simulink model "SNS_Li_CPG"  (R2025a)
settings: Solver=ode45  StartTime=0.0  StopTime=30  MaxStep=1e-3  RelTol=1e-3
libraries: SNS_Library x134
settings Model: Creator=Ben Bolen  LastModifiedBy=Ben Bolen

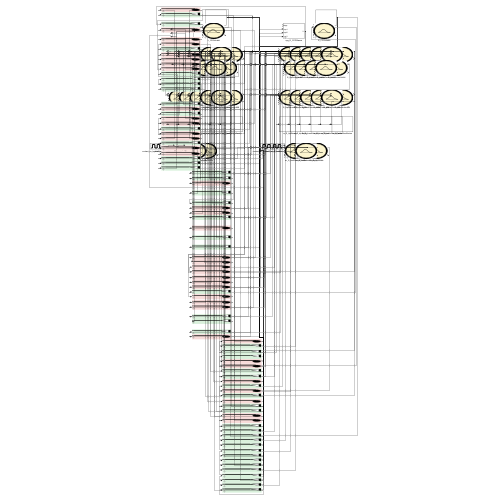
[thumbnail: Simulink's stored preview of the top-level diagram]
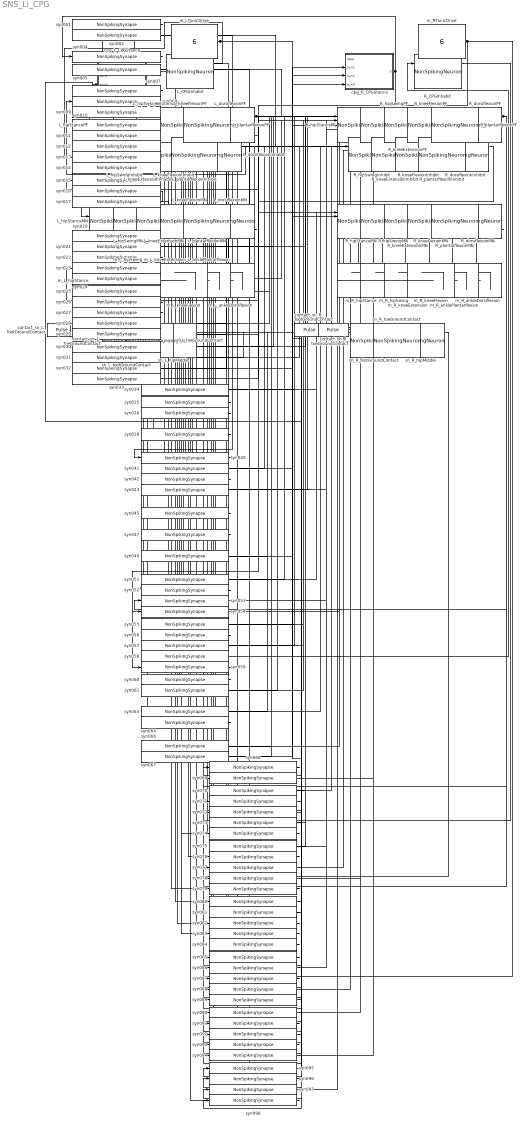
== system SNS_Li_CPG ==
  L_CPGInhabit : SNS_Library/NonSpikingNeuron  Vrest=-52  Gm=0.12  Cm=5  Thr=-50  Slope=1
  L_dorsiflexionInhabit : SNS_Library/NonSpikingNeuron  Vrest=-52  Gm=0.12  Cm=5  Thr=-50  Slope=1
  L_dorsiflexionMN : SNS_Library/NonSpikingNeuron  Vrest=-52  Gm=0.5  Cm=5  Thr=-45  Slope=1
  L_dorsiflexionPF : SNS_Library/NonSpikingNeuron  Vrest=-52  Gm=0.12  Cm=5  Thr=-50  Slope=1
  L_hipStanceMN : SNS_Library/NonSpikingNeuron  Vrest=-52  Gm=0.5  Cm=5  Thr=-45  Slope=1
  L_hipStancePF : SNS_Library/NonSpikingNeuron  Vrest=-52  Gm=0.12  Cm=5  Thr=-50  Slope=1
  L_hipSwingInhibit : SNS_Library/NonSpikingNeuron  Vrest=-52  Gm=0.12  Cm=5  Thr=-50  Slope=1
  L_hipSwingMN : SNS_Library/NonSpikingNeuron  Vrest=-52  Gm=0.5  Cm=5  Thr=-45  Slope=1
  L_hipSwingPF : SNS_Library/NonSpikingNeuron  Vrest=-52  Gm=0.12  Cm=5  Thr=-50  Slope=1
  L_kneeExtensionInhabit : SNS_Library/NonSpikingNeuron  Vrest=-52  Gm=0.12  Cm=5  Thr=-50  Slope=1
  L_kneeExtensionMN : SNS_Library/NonSpikingNeuron  Vrest=-52  Gm=0.5  Cm=5  Thr=-45  Slope=1
  L_kneeExtensionPF : SNS_Library/NonSpikingNeuron  Vrest=-52  Gm=0.12  Cm=5  Thr=-50  Slope=1
  L_kneeFlexionInhibit : SNS_Library/NonSpikingNeuron  Vrest=-52  Gm=0.12  Cm=5  Thr=-50  Slope=1
  L_kneeFlexionMN : SNS_Library/NonSpikingNeuron  Vrest=-52  Gm=0.5  Cm=5  Thr=-45  Slope=1
  L_kneeFlexionPF : SNS_Library/NonSpikingNeuron  Vrest=-52  Gm=0.12  Cm=5  Thr=-50  Slope=1
  L_plantarflexionInhibit : SNS_Library/NonSpikingNeuron  Vrest=-52  Gm=0.12  Cm=5  Thr=-50  Slope=1
  L_plantarflexionMN : SNS_Library/NonSpikingNeuron  Vrest=-52  Gm=0.5  Cm=5  Thr=-45  Slope=1
  L_plantarflexionPF : SNS_Library/NonSpikingNeuron  Vrest=-52  Gm=0.12  Cm=5  Thr=-50  Slope=1
  R_CPGInhabit : SNS_Library/NonSpikingNeuron  Vrest=-52  Gm=0.12  Cm=5  Thr=-50  Slope=1
  R_dorsiflexionInhibit : SNS_Library/NonSpikingNeuron  Vrest=-52  Gm=0.12  Cm=5  Thr=-50  Slope=1
  R_dorsiflexionMN : SNS_Library/NonSpikingNeuron  Vrest=-52  Gm=0.5  Cm=5  Thr=-45  Slope=1
  R_dorsiflexionPF : SNS_Library/NonSpikingNeuron  Vrest=-52  Gm=0.12  Cm=5  Thr=-50  Slope=1
  R_hipStanceMN : SNS_Library/NonSpikingNeuron  Vrest=-52  Gm=0.5  Cm=5  Thr=-45  Slope=1
  R_hipStancePF : SNS_Library/NonSpikingNeuron  Vrest=-52  Gm=0.12  Cm=5  Thr=-50  Slope=1
  R_hipSwingInhibit : SNS_Library/NonSpikingNeuron  Vrest=-52  Gm=0.12  Cm=5  Thr=-50  Slope=1
  R_hipSwingMN : SNS_Library/NonSpikingNeuron  Vrest=-52  Gm=0.5  Cm=5  Thr=-45  Slope=1
  R_hipSwingPF : SNS_Library/NonSpikingNeuron  Vrest=-52  Gm=0.12  Cm=5  Thr=-50  Slope=1
  R_kneeExtensionInhibit : SNS_Library/NonSpikingNeuron  Vrest=-52  Gm=0.12  Cm=5  Thr=-50  Slope=1
  R_kneeExtensionMN : SNS_Library/NonSpikingNeuron  Vrest=-52  Gm=0.5  Cm=5  Thr=-45  Slope=1
  R_kneeExtensionPF : SNS_Library/NonSpikingNeuron  Vrest=-52  Gm=0.12  Cm=5  Thr=-50  Slope=1
  R_kneeFlexionInhibit : SNS_Library/NonSpikingNeuron  Vrest=-52  Gm=0.12  Cm=5  Thr=-50  Slope=1
  R_kneeFlexionMN : SNS_Library/NonSpikingNeuron  Vrest=-52  Gm=0.5  Cm=5  Thr=-45  Slope=1
  R_kneeFlexionPF : SNS_Library/NonSpikingNeuron  Vrest=-52  Gm=0.12  Cm=5  Thr=-50  Slope=1
  R_plantarflexionInhibit : SNS_Library/NonSpikingNeuron  Vrest=-52  Gm=0.12  Cm=5  Thr=-50  Slope=1
  R_plantarflexionMN : SNS_Library/NonSpikingNeuron  Vrest=-52  Gm=0.5  Cm=5  Thr=-45  Slope=1
  R_plantarflexionPF : SNS_Library/NonSpikingNeuron  Vrest=-52  Gm=0.12  Cm=5  Thr=-50  Slope=1
  contact_sn_L_footGroundContact : DiscretePulseGenerator  PulseType=Time based  Amplitude=10  PulseWidth=35
  contact_sn_L_toeGroundContact : DiscretePulseGenerator  PulseType=Time based  Amplitude=10  PulseWidth=35
  contact_sn_R_footGroundContact : DiscretePulseGenerator  PulseType=Time based  Amplitude=10  PulseWidth=35  PhaseDelay=1
  contact_sn_R_toeGroundContact : DiscretePulseGenerator  PulseType=Time based  Amplitude=10  PulseWidth=35  PhaseDelay=1
  cpg_L_CPGStance : Subsystem
      mask help: Li stance CPG v1 (ADAPTATION): graded cell + slow Adp burst termination, tau = documented tau_Ca 7.5 s. Ports: 1 Iapp (nA currents), 2-4 synaptic inputs, out = cell V (mV).
  cpg_R_CPGStance : Subsystem
      mask help: Li stance CPG v1 (ADAPTATION): graded cell + slow Adp burst termination, tau = documented tau_Ca 7.5 s. Ports: 1 Iapp (nA currents), 2-4 synaptic inputs, out = cell V (mV).
  in_LTonicDrive : Constant  Value=6
  in_RTonicDrive : Constant  Value=6
  m_L_ankleDorsiflexion : Terminator
  m_L_anklePlantarflexion : Terminator
  m_L_hipStance : Terminator
  m_L_hipSwing : Terminator
  m_L_kneeExtension : Terminator
  m_L_kneeFlexion : Terminator
  m_R_ankleDorsiflexion : Terminator
  m_R_anklePlantarflexion : Terminator
  m_R_hipStance : Terminator
  m_R_hipSwing : Terminator
  m_R_kneeExtension : Terminator
  m_R_kneeFlexion : Terminator
  sn_L_footGroundContact : SNS_Library/NonSpikingNeuron  Vrest=-52  Gm=0.12  Cm=2  Thr=-55  Slope=1
  sn_L_hipMiddle : SNS_Library/NonSpikingNeuron  Vrest=-52  Gm=0.12  Cm=5  Thr=-50  Slope=1
  sn_L_toeGroundContact : SNS_Library/NonSpikingNeuron  Vrest=-52  Gm=0.12  Cm=2  Thr=-55  Slope=1
  sn_R_footGroundContact : SNS_Library/NonSpikingNeuron  Vrest=-52  Gm=0.12  Cm=2  Thr=-55  Slope=1
  sn_R_hipMiddle : SNS_Library/NonSpikingNeuron  Vrest=-52  Gm=0.12  Cm=5  Thr=-50  Slope=1
  sn_R_toeGroundContact : SNS_Library/NonSpikingNeuron  Vrest=-52  Gm=0.12  Cm=2  Thr=-55  Slope=1
  syn001 : SNS_Library/NonSpikingSynapse  gmax=1  Esyn=-72  ThrPre=-50  SlopePre=1
  syn002 : SNS_Library/NonSpikingSynapse  gmax=8  Esyn=0  ThrPre=-50  SlopePre=1
  syn004 : SNS_Library/NonSpikingSynapse  gmax=1  Esyn=0  ThrPre=-50  SlopePre=1
  syn005 : SNS_Library/NonSpikingSynapse  gmax=1  Esyn=-72  ThrPre=-50  SlopePre=1
  syn007 : SNS_Library/NonSpikingSynapse  gmax=1  Esyn=-72  ThrPre=-50  SlopePre=1
  syn008 : SNS_Library/NonSpikingSynapse  gmax=1  Esyn=-72  ThrPre=-50  SlopePre=1
  syn009 : SNS_Library/NonSpikingSynapse  gmax=1  Esyn=0  ThrPre=-50  SlopePre=1
  syn010 : SNS_Library/NonSpikingSynapse  gmax=1  Esyn=-72  ThrPre=-50  SlopePre=1
  syn011 : SNS_Library/NonSpikingSynapse  gmax=1  Esyn=-72  ThrPre=-50  SlopePre=1
  syn012 : SNS_Library/NonSpikingSynapse  gmax=1  Esyn=-72  ThrPre=-50  SlopePre=1
  syn013 : SNS_Library/NonSpikingSynapse  gmax=1  Esyn=-72  ThrPre=-50  SlopePre=1
  syn014 : SNS_Library/NonSpikingSynapse  gmax=8  Esyn=0  ThrPre=-50  SlopePre=1
  syn015 : SNS_Library/NonSpikingSynapse  gmax=1  Esyn=0  ThrPre=-50  SlopePre=1
  syn016 : SNS_Library/NonSpikingSynapse  gmax=1  Esyn=0  ThrPre=-50  SlopePre=1
  syn017 : SNS_Library/NonSpikingSynapse  gmax=1  Esyn=0  ThrPre=-50  SlopePre=1
  syn020 : SNS_Library/NonSpikingSynapse  gmax=1  Esyn=0  ThrPre=-50  SlopePre=1
  syn021 : SNS_Library/NonSpikingSynapse  gmax=1  Esyn=-72  ThrPre=-50  SlopePre=1
  syn022 : SNS_Library/NonSpikingSynapse  gmax=1  Esyn=0  ThrPre=-50  SlopePre=1
  syn023 : SNS_Library/NonSpikingSynapse  gmax=1  Esyn=-72  ThrPre=-50  SlopePre=1
  syn024 : SNS_Library/NonSpikingSynapse  gmax=1  Esyn=-72  ThrPre=-50  SlopePre=1
  syn025 : SNS_Library/NonSpikingSynapse  gmax=1  Esyn=0  ThrPre=-50  SlopePre=1
  syn026 : SNS_Library/NonSpikingSynapse  gmax=1  Esyn=-72  ThrPre=-50  SlopePre=1
  syn027 : SNS_Library/NonSpikingSynapse  gmax=1  Esyn=-72  ThrPre=-50  SlopePre=1
  syn028 : SNS_Library/NonSpikingSynapse  gmax=2  Esyn=0  ThrPre=-50  SlopePre=1
  syn029 : SNS_Library/NonSpikingSynapse  gmax=1  Esyn=-72  ThrPre=-50  SlopePre=1
  syn030 : SNS_Library/NonSpikingSynapse  gmax=1  Esyn=-72  ThrPre=-50  SlopePre=1
  syn031 : SNS_Library/NonSpikingSynapse  gmax=5  Esyn=0  ThrPre=-50  SlopePre=1
  syn032 : SNS_Library/NonSpikingSynapse  gmax=1  Esyn=0  ThrPre=-50  SlopePre=1
  syn033 : SNS_Library/NonSpikingSynapse  gmax=1  Esyn=0  ThrPre=-50  SlopePre=1
  syn034 : SNS_Library/NonSpikingSynapse  gmax=1  Esyn=0  ThrPre=-50  SlopePre=1
  syn035 : SNS_Library/NonSpikingSynapse  gmax=1  Esyn=0  ThrPre=-50  SlopePre=1
  syn036 : SNS_Library/NonSpikingSynapse  gmax=1  Esyn=-72  ThrPre=-50  SlopePre=1
  syn038 : SNS_Library/NonSpikingSynapse  gmax=5  Esyn=0  ThrPre=-50  SlopePre=1
  syn040 : SNS_Library/NonSpikingSynapse  gmax=8  Esyn=0  ThrPre=-50  SlopePre=1
  syn041 : SNS_Library/NonSpikingSynapse  gmax=1  Esyn=-72  ThrPre=-50  SlopePre=1
  syn042 : SNS_Library/NonSpikingSynapse  gmax=1  Esyn=-72  ThrPre=-50  SlopePre=1
  syn043 : SNS_Library/NonSpikingSynapse  gmax=1  Esyn=0  ThrPre=-50  SlopePre=1
  syn045 : SNS_Library/NonSpikingSynapse  gmax=1  Esyn=-72  ThrPre=-50  SlopePre=1
  syn047 : SNS_Library/NonSpikingSynapse  gmax=6  Esyn=0  ThrPre=-50  SlopePre=1
  syn049 : SNS_Library/NonSpikingSynapse  gmax=4  Esyn=0  ThrPre=-50  SlopePre=1
  syn051 : SNS_Library/NonSpikingSynapse  gmax=1  Esyn=-72  ThrPre=-50  SlopePre=1
  syn052 : SNS_Library/NonSpikingSynapse  gmax=1  Esyn=-72  ThrPre=-50  SlopePre=1
  syn053 : SNS_Library/NonSpikingSynapse  gmax=1  Esyn=-72  ThrPre=-50  SlopePre=1
  syn054 : SNS_Library/NonSpikingSynapse  gmax=1  Esyn=-72  ThrPre=-50  SlopePre=1
  syn055 : SNS_Library/NonSpikingSynapse  gmax=1  Esyn=-72  ThrPre=-50  SlopePre=1
  syn056 : SNS_Library/NonSpikingSynapse  gmax=1  Esyn=-72  ThrPre=-50  SlopePre=1
  syn057 : SNS_Library/NonSpikingSynapse  gmax=1  Esyn=-72  ThrPre=-50  SlopePre=1
  syn058 : SNS_Library/NonSpikingSynapse  gmax=6  Esyn=0  ThrPre=-50  SlopePre=1
  syn059 : SNS_Library/NonSpikingSynapse  gmax=1  Esyn=-72  ThrPre=-50  SlopePre=1
  syn060 : SNS_Library/NonSpikingSynapse  gmax=1  Esyn=-72  ThrPre=-50  SlopePre=1
  syn061 : SNS_Library/NonSpikingSynapse  gmax=1  Esyn=-72  ThrPre=-50  SlopePre=1
  syn063 : SNS_Library/NonSpikingSynapse  gmax=6  Esyn=0  ThrPre=-50  SlopePre=1
  syn064 : SNS_Library/NonSpikingSynapse  gmax=1  Esyn=0  ThrPre=-50  SlopePre=1
  syn066 : SNS_Library/NonSpikingSynapse  gmax=1  Esyn=0  ThrPre=-50  SlopePre=1
  syn067 : SNS_Library/NonSpikingSynapse  gmax=1  Esyn=-72  ThrPre=-50  SlopePre=1
  syn068 : SNS_Library/NonSpikingSynapse  gmax=1  Esyn=-72  ThrPre=-50  SlopePre=1
  syn069 : SNS_Library/NonSpikingSynapse  gmax=1  Esyn=0  ThrPre=-50  SlopePre=1
  syn070 : SNS_Library/NonSpikingSynapse  gmax=8  Esyn=0  ThrPre=-50  SlopePre=1
  syn071 : SNS_Library/NonSpikingSynapse  gmax=1  Esyn=0  ThrPre=-50  SlopePre=1
  syn072 : SNS_Library/NonSpikingSynapse  gmax=1  Esyn=-72  ThrPre=-50  SlopePre=1
  syn073 : SNS_Library/NonSpikingSynapse  gmax=1  Esyn=-72  ThrPre=-50  SlopePre=1
  syn074 : SNS_Library/NonSpikingSynapse  gmax=8  Esyn=0  ThrPre=-50  SlopePre=1
  syn075 : SNS_Library/NonSpikingSynapse  gmax=1  Esyn=0  ThrPre=-50  SlopePre=1
  syn076 : SNS_Library/NonSpikingSynapse  gmax=1  Esyn=-72  ThrPre=-50  SlopePre=1
  syn077 : SNS_Library/NonSpikingSynapse  gmax=8  Esyn=0  ThrPre=-50  SlopePre=1
  syn078 : SNS_Library/NonSpikingSynapse  gmax=1  Esyn=-72  ThrPre=-50  SlopePre=1
  syn079 : SNS_Library/NonSpikingSynapse  gmax=2  Esyn=0  ThrPre=-50  SlopePre=1
  syn080 : SNS_Library/NonSpikingSynapse  gmax=1  Esyn=-72  ThrPre=-50  SlopePre=1
  syn081 : SNS_Library/NonSpikingSynapse  gmax=6  Esyn=0  ThrPre=-50  SlopePre=1
  syn082 : SNS_Library/NonSpikingSynapse  gmax=4  Esyn=0  ThrPre=-50  SlopePre=1
  syn083 : SNS_Library/NonSpikingSynapse  gmax=1  Esyn=-72  ThrPre=-50  SlopePre=1
  syn084 : SNS_Library/NonSpikingSynapse  gmax=1  Esyn=-72  ThrPre=-50  SlopePre=1
  syn085 : SNS_Library/NonSpikingSynapse  gmax=5  Esyn=0  ThrPre=-50  SlopePre=1
  syn086 : SNS_Library/NonSpikingSynapse  gmax=5  Esyn=0  ThrPre=-50  SlopePre=1
  syn087 : SNS_Library/NonSpikingSynapse  gmax=5  Esyn=0  ThrPre=-50  SlopePre=1
  syn088 : SNS_Library/NonSpikingSynapse  gmax=5  Esyn=0  ThrPre=-50  SlopePre=1
  syn089 : SNS_Library/NonSpikingSynapse  gmax=6  Esyn=0  ThrPre=-50  SlopePre=1
  syn090 : SNS_Library/NonSpikingSynapse  gmax=5  Esyn=0  ThrPre=-50  SlopePre=1
  syn091 : SNS_Library/NonSpikingSynapse  gmax=5  Esyn=0  ThrPre=-50  SlopePre=1
  syn092 : SNS_Library/NonSpikingSynapse  gmax=6  Esyn=0  ThrPre=-50  SlopePre=1
  syn093 : SNS_Library/NonSpikingSynapse  gmax=6  Esyn=0  ThrPre=-50  SlopePre=1
  syn094 : SNS_Library/NonSpikingSynapse  gmax=5  Esyn=0  ThrPre=-50  SlopePre=1
  syn095 : SNS_Library/NonSpikingSynapse  gmax=5  Esyn=0  ThrPre=-50  SlopePre=1
  syn096 : SNS_Library/NonSpikingSynapse  gmax=6  Esyn=0  ThrPre=-50  SlopePre=1
  syn097 : SNS_Library/NonSpikingSynapse  gmax=5  Esyn=0  ThrPre=-50  SlopePre=1
  syn098 : SNS_Library/NonSpikingSynapse  gmax=5  Esyn=0  ThrPre=-50  SlopePre=1
  wires:
  contact_sn_L_footGroundContact/1 -> sn_L_footGroundContact/1
  contact_sn_L_toeGroundContact/1 -> sn_L_toeGroundContact/1
  contact_sn_R_footGroundContact/1 -> sn_R_footGroundContact/1
  contact_sn_R_toeGroundContact/1 -> sn_R_toeGroundContact/1
  L_hipStancePF/1 -> syn001/1, syn016/1, syn027/1, syn079/1
  syn001/1 -> L_hipSwingPF/2
  sn_R_footGroundContact/1 -> syn002/1, syn049/1, syn063/1, syn081/1
  syn002/1 -> R_kneeFlexionInhibit/2
  R_kneeFlexionMN/2 -> m_R_kneeFlexion/1
  cpg_R_CPGStance/1(V) -> syn004/1, syn023/1, syn071/1
  syn004/1 -> L_hipSwingPF/3
  R_kneeExtensionPF/1 -> syn005/1, syn025/1, syn051/1
  syn005/1 -> R_kneeFlexionPF/2
  R_plantarflexionMN/2 -> m_R_anklePlantarflexion/1
  L_kneeExtensionPF/1 -> syn007/1, syn035/1, syn036/1
  syn007/1 -> L_kneeFlexionPF/2
  L_dorsiflexionInhabit/1 -> syn008/1
  syn008/1 -> L_dorsiflexionPF/2
  L_kneeFlexionPF/1 -> syn009/1, syn026/1, syn060/1
  syn009/1 -> L_kneeFlexionMN/2
  L_hipSwingPF/1 -> syn010/1, syn022/1, syn064/1, syn074/1, syn083/1
  syn010/1 -> L_hipStanceMN/2
  R_hipStancePF/1 -> syn011/1, syn028/1, syn029/1, syn032/1
  syn011/1 -> R_hipSwingPF/2
  R_plantarflexionInhibit/1 -> syn012/1
  syn012/1 -> R_plantarflexionPF/2
  L_CPGInhabit/1 -> syn013/1
  syn013/1 -> cpg_L_CPGStance/2(syn1)
  sn_L_footGroundContact/1 -> syn014/1, syn047/1, syn058/1, syn082/1
  syn014/1 -> L_kneeFlexionInhibit/2
  L_dorsiflexionPF/1 -> syn015/1, syn059/1, syn068/1
  syn015/1 -> L_dorsiflexionMN/2
  syn016/1 -> L_hipStanceMN/3
  L_plantarflexionPF/1 -> syn017/1, syn045/1, syn056/1
  syn017/1 -> L_plantarflexionMN/2
  L_hipStanceMN/2 -> m_L_hipStance/1
  L_plantarflexionMN/2 -> m_L_anklePlantarflexion/1
  cpg_L_CPGStance/1(V) -> syn020/1, syn033/1, syn080/1
  syn020/1 -> L_hipStancePF/2
  R_plantarflexionPF/1 -> syn021/1, syn030/1, syn043/1
  syn021/1 -> R_dorsiflexionPF/2
  syn022/1 -> L_hipSwingMN/2
  syn023/1 -> cpg_L_CPGStance/3(syn2)
  R_kneeFlexionInhibit/1 -> syn024/1
  syn024/1 -> R_kneeFlexionPF/3
  syn025/1 -> R_kneeExtensionMN/2
  syn026/1 -> L_kneeExtensionPF/2
  syn027/1 -> L_hipSwingMN/3
  syn028/1 -> R_kneeExtensionPF/2
  syn029/1 -> R_hipSwingMN/2
  syn030/1 -> R_dorsiflexionMN/2
  sn_R_toeGroundContact/1 -> syn031/1
  syn031/1 -> R_dorsiflexionInhibit/2
  syn032/1 -> R_hipStanceMN/2
  syn033/1 -> R_hipSwingPF/3
  R_kneeFlexionPF/1 -> syn034/1, syn055/1, syn057/1
  syn034/1 -> R_kneeFlexionMN/2
  syn035/1 -> L_kneeExtensionMN/2
  syn036/1 -> L_kneeFlexionMN/3
  L_kneeFlexionMN/2 -> m_L_kneeFlexion/1
  sn_L_toeGroundContact/1 -> syn038/1
  syn038/1 -> L_dorsiflexionInhabit/2
  L_dorsiflexionMN/2 -> m_L_ankleDorsiflexion/1
  sn_L_hipMiddle/1 -> syn040/1
  syn040/1 -> L_kneeFlexionInhibit/3
  R_hipSwingInhibit/1 -> syn041/1
  syn041/1 -> R_hipSwingPF/4
  L_kneeFlexionInhibit/1 -> syn042/1
  syn042/1 -> L_kneeFlexionPF/3
  syn043/1 -> R_plantarflexionMN/2
  R_hipStanceMN/2 -> m_R_hipStance/1
  syn045/1 -> L_dorsiflexionPF/3
  L_kneeExtensionMN/2 -> m_L_kneeExtension/1
  syn047/1 -> L_plantarflexionInhibit/2
  R_hipSwingMN/2 -> m_R_hipSwing/1
  syn049/1 -> R_hipSwingInhibit/2
  R_kneeExtensionMN/2 -> m_R_kneeExtension/1
  syn051/1 -> R_kneeFlexionMN/3
  L_hipSwingInhibit/1 -> syn052/1
  syn052/1 -> L_hipSwingPF/4
  R_dorsiflexionPF/1 -> syn053/1, syn069/1, syn078/1
  syn053/1 -> R_plantarflexionPF/3
  R_dorsiflexionInhibit/1 -> syn054/1
  syn054/1 -> R_dorsiflexionPF/3
  syn055/1 -> R_kneeExtensionPF/3
  syn056/1 -> L_dorsiflexionMN/3
  syn057/1 -> R_kneeExtensionMN/3
  syn058/1 -> R_CPGInhabit/2
  syn059/1 -> L_plantarflexionPF/2
  syn060/1 -> L_kneeExtensionMN/3
  R_kneeExtensionInhibit/1 -> syn061/1
  syn061/1 -> R_kneeExtensionPF/4
  L_hipSwingMN/2 -> m_L_hipSwing/1
  syn063/1 -> R_plantarflexionInhibit/2
  syn064/1 -> L_dorsiflexionPF/4
  R_dorsiflexionMN/2 -> m_R_ankleDorsiflexion/1
  R_hipSwingPF/1 -> syn066/1, syn067/1, syn070/1, syn073/1, syn075/1
  syn066/1 -> R_dorsiflexionPF/4
  syn067/1 -> R_hipStancePF/2
  syn068/1 -> L_plantarflexionMN/3
  syn069/1 -> R_dorsiflexionMN/3
  syn070/1 -> R_kneeExtensionInhibit/2
  syn071/1 -> R_hipStancePF/3
  R_CPGInhabit/1 -> syn072/1
  syn072/1 -> cpg_R_CPGStance/2(syn1)
  syn073/1 -> R_hipStanceMN/3
  syn074/1 -> L_kneeExtensionInhabit/2
  syn075/1 -> R_hipSwingMN/3
  L_kneeExtensionInhabit/1 -> syn076/1
  syn076/1 -> L_kneeExtensionPF/3
  sn_R_hipMiddle/1 -> syn077/1
  syn077/1 -> R_kneeFlexionInhibit/3
  syn078/1 -> R_plantarflexionMN/3
  syn079/1 -> L_kneeExtensionPF/4
  syn080/1 -> cpg_R_CPGStance/3(syn2)
  syn081/1 -> L_CPGInhabit/2
  syn082/1 -> L_hipSwingInhibit/2
  syn083/1 -> L_hipStancePF/3
  L_plantarflexionInhibit/1 -> syn084/1
  syn084/1 -> L_plantarflexionPF/3
  in_LTonicDrive/1 -> syn085/1, syn087/1, syn091/1, syn092/1, syn093/1, syn096/1, syn098/1
  syn085/1 -> L_hipSwingPF/5
  in_RTonicDrive/1 -> syn086/1, syn088/1, syn089/1, syn090/1, syn094/1, syn095/1, syn097/1
  syn086/1 -> R_hipSwingPF/5
  syn087/1 -> L_kneeFlexionPF/4
  syn088/1 -> R_kneeFlexionPF/4
  syn089/1 -> cpg_R_CPGStance/4(syn3)
  syn090/1 -> R_plantarflexionPF/4
  syn091/1 -> L_kneeExtensionPF/5
  syn092/1 -> cpg_L_CPGStance/4(syn3)
  syn093/1 -> L_plantarflexionPF/4
  syn094/1 -> R_dorsiflexionPF/5
  syn095/1 -> R_hipStancePF/4
  syn096/1 -> L_dorsiflexionPF/5
  syn097/1 -> R_kneeExtensionPF/5
  syn098/1 -> L_hipStancePF/4

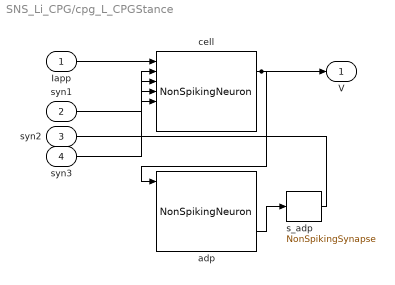
== system SNS_Li_CPG/cpg_L_CPGStance ==
  Iapp : Inport
  syn1 : Inport  Port=2
  syn2 : Inport  Port=3
  syn3 : Inport  Port=4
  adp : SNS_Library/NonSpikingNeuron  Vrest=-52  Gm=0.1  Cm=750  Thr=-45  Slope=1
  cell : SNS_Library/NonSpikingNeuron  Vrest=-52  Gm=0.5  Cm=5  Thr=-45  Slope=1
  s_adp : SNS_Library/NonSpikingSynapse  gmax=0.5  Esyn=-72  ThrPre=-45  SlopePre=1
  V : Outport
  wires:
  Iapp/1 -> cell/1
  cell/1 -> V/1, adp/1
  adp/2 -> s_adp/1
  s_adp/1 -> cell/2
  syn1/1 -> cell/3
  syn2/1 -> cell/4
  syn3/1 -> cell/5

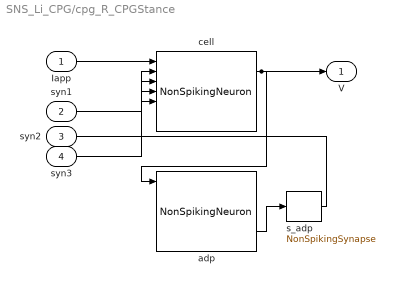
== system SNS_Li_CPG/cpg_R_CPGStance ==
  Iapp : Inport
  syn1 : Inport  Port=2
  syn2 : Inport  Port=3
  syn3 : Inport  Port=4
  adp : SNS_Library/NonSpikingNeuron  Vrest=-52  Gm=0.1  Cm=750  Thr=-45  Slope=1
  cell : SNS_Library/NonSpikingNeuron  Vrest=-52  Gm=0.5  Cm=5  Thr=-45  Slope=1
  s_adp : SNS_Library/NonSpikingSynapse  gmax=0.5  Esyn=-72  ThrPre=-45  SlopePre=1
  V : Outport
  wires:
  Iapp/1 -> cell/1
  cell/1 -> V/1, adp/1
  adp/2 -> s_adp/1
  s_adp/1 -> cell/2
  syn1/1 -> cell/3
  syn2/1 -> cell/4
  syn3/1 -> cell/5
